simulink model "PMSM_MC_2025a"  (R2025a)
settings: Solver=FixedStepDiscrete  StartTime=0.0  StopTime=10.0  FixedStep=0.00005  RelTol=1e-3
values from neighbouring files (symbols this model uses):
  MC_DCurrLopKi_CFG = 0.008293758    [PMSM_MC_Data_2025a.sldd]
  MC_DCurrLopKp_CFG = 0.0870848    [PMSM_MC_Data_2025a.sldd]
  MC_MotModeDebug_CFG = 255.0    [PMSM_MC_Data_2025a.sldd]
  MC_POLE_NUM_CFG = 7.0    [PMSM_MC_Data_2025a.sldd]
  MC_QCurrLopKi_CFG = 0.008293758    [PMSM_MC_Data_2025a.sldd]
  MC_QCurrLopKp_CFG = 0.0870848    [PMSM_MC_Data_2025a.sldd]
  MC_SpdLopKi_CFG = 1.0E-5    [PMSM_MC_Data_2025a.sldd]
  MC_SpdLopKp_CFG = 0.002    [PMSM_MC_Data_2025a.sldd]
  OpenLoopEn_CFG = 0.0    [PMSM_MC_Data_2025a.sldd]
  SensorLessEn_CFG = 0.0    [PMSM_MC_Data_2025a.sldd]
  SensorLessType_CFG = 1.0    [PMSM_MC_Data_2025a.sldd]
undefined symbols (not defined in the file or in its folder): Ls, magnitude, Rs
libraries: simulink x25, slpidlib x6
(part 3 of 3)

== stateflow chart PMSM_MC_2025a/PMSM_MC/MC_HighFrqTask/OpenLopMod/OpenLopThetaeCal ==
  state Stop
    en:
    //init output
    Thetae_SensLess = 0;
    OLStartCompletedFlag = 0;
    TransmActiveFlag = 0;
    SL_TransferActive = 0;
    //init local variable
    WeRefRamped = 0;
    Thetae_OL = 0;
    OLStableCnt = 0;
    Blend = 0.0F;
    TransmStep = 0;
    TransmFactor = 0;
    DeltaStep  = 0;
    Err = 0;
    RawNow = 0;
    note: 注意要给局部变量
        | 初始化赋值处理
  state VFOpenLoop
    state Align
      en:
      Thetae_SensLess = 0;
    state Open
      en,du:
      Ramping(OLWeRef,OLWeRampMaxStep);
      OLThetaeSum();
      Thetae_SensLess = Thetae_OL;
    (default) -> VFOpenLoop.Align
    VFOpenLoop.Align -> VFOpenLoop.Open : [after(100,msec)]
  state IFStart
    state Align
      en:
      Thetae_SensLess = 0;
    state Open
      en,du:
      Ramping(OLWeRef,OLWeRampMaxStep);
      OLThetaeSum();
      OLStableCntSum();
      Thetae_SensLess = Thetae_OL;
    note: TransmStep其实是根据切换时间算每次
        | 权重增加的步长，最终完成切换从0->1
    state Transm
      en:
      //相位计算与方向判断
      TransmActiveFlag = 1;
      SL_TransferActive = 1;
      Blend  = 0;
      TransmFactor = 0.0F;
      //cal steps according time
      TransmStep = Ts * 1000.0F / OLWeightedTransmTime;
      //transmite from open to close
      WeightedTransmite();
      du:
      WeightedTransmite();
    (default) -> IFStart.Align
    IFStart.Align -> IFStart.Open : [after(100,msec)]
    IFStart.Open -> Transm : [OLStableCnt>OLSpdStableCnt && SL_SpeedReady]
  state Ramping(in,MaxStep) [function]
    note: WeRefRamped指当前的局部真实被电机使用的一个设定递增速度值，电机最开始为0，当我的速度期望值比较大的时候，就会与现在WeRefRamped真实速度设定值比较，让他以MaxStep的递增速度累加或者累减，直到设定值与期望值的差值在[-MaxStep,+MaxStep]时，将当前速度赋值给定成期望值
    (default) -> (junction 23)
    (junction 23) -> (junction 30) [order 1] : [in - WeRefRamped > MaxStep]
    (junction 23) -> (junction 32) [order 2]
    (junction 30) -> (junction 41) : {
        | WeRefRamped = WeRefRamped + MaxStep;
        | }
    (junction 32) -> (junction 34) [order 1] : [in - WeRefRamped < -MaxStep]
    (junction 32) -> (junction 36) [order 2] : {
        | WeRefRamped = in;
        | }
    (junction 34) -> (junction 38) : {
        | WeRefRamped = WeRefRamped - MaxStep;
        | }
    (junction 38) -> (junction 36)
    (junction 41) -> (junction 38)
    (junction 36) -> (junction 43)
  state OLThetaeSum [function]
    note: MotCtrMode==8条件是为了VF开环使用的，
        | 我们的VF开环只进行正向累加，而MotorSpdRef
        | 主要用于IF启动的时候使用
    (default) -> (junction 28)
    (junction 28) -> (junction 48) [order 1] : [MotorSpdRef > 0||...
        | MotCtrMode == 8]
    (junction 28) -> (junction 52) [order 2] : {
        | Thetae_OL = Thetae_OL - WeRefRamped*Ts;
        | }
    (junction 48) -> (junction 50) : {
        | Thetae_OL = Thetae_OL + WeRefRamped*Ts;
        | }
    (junction 50) -> (junction 52)
    (junction 52) -> (junction 55)
    (junction 55) -> (junction 57) [order 1] : [Thetae_OL < 0]
    (junction 55) -> (junction 59) [order 2] : {
        | //set range to [0 2pi]
        | Thetae_OL = fmod(Thetae_OL,6.28318531F);
        | }
    (junction 57) -> (junction 58) : {
        | //set range to [0 2pi]
        | Thetae_OL  = -Thetae_OL;
        | Thetae_OL = fmod(Thetae_OL,6.28318531F);
        | Thetae_OL =  6.28318531F - Thetae_OL;
        | }
    (junction 58) -> (junction 59)
    (junction 59) -> (junction 60)
  state OLStableCntSum [function]
    note: 如果观测器速度大于设定的稳定速度就开始稳定计次
        | 如果出现速度小于阈值则计次再次为0
    (default) -> (junction 79)
    (junction 79) -> (junction 87) [order 1] : [(MotorSpdRef > 0 && We_Est>OLSpdStableThd) ||...
        | (MotorSpdRef < 0 && We_Est<-OLSpdStableThd)]
    (junction 87) -> (junction 85) [order 2]
    (junction 79) -> (junction 85) [order 2] : {
        | OLStableCnt = 0;
        | }
    (junction 87) -> (junction 711) [order 1] : [OLStableCnt <= OLSpdStableCnt]
    (junction 711) -> (junction 86) : {
        | OLStableCnt++;
        | }
    (junction 86) -> (junction 85)
    (junction 85) -> (junction 88)
  state WeightedTransmite_origin [function] [commented out]
    (default) -> (junction 279) [commented out] : {
        | //update factor each sw cycle
        | %TransmFactor = TransmFactor+TransmStep;
        | //open loop angle calculate
        | Ramping(OLWeRef,OLWeRampMaxStep);
        | OLThetaeSum();
        | RawNow = Thetae_Est -Thetae_OL;
        |
        | }
    (junction 279) -> (junction 281) [commented out] : [RawNow>3.1415927F]
    (junction 279) -> (junction 285) [commented out]
    (junction 281) -> (junction 283) [commented out] : {
        | RawNow = RawNow - 6.2831855F;
        | }
    (junction 283) -> (junction 285) [commented out]
    (junction 285) -> (junction 288) [commented out]
    (junction 288) -> (junction 290) [commented out] : [RawNow<-3.1415927F]
    (junction 288) -> (junction 294) [commented out]
    (junction 290) -> (junction 292) [commented out] : {
        | RawNow = RawNow + 6.2831855F;
        | }
    (junction 292) -> (junction 294) [commented out]
    (junction 294) -> (junction 300) [commented out] : {
        | Err = RawNow - PhaseOffset;
        | }
    (junction 300) -> (junction 310) [commented out] : [Err>3.1415927F]
    (junction 300) -> (junction 309) [commented out]
    (junction 310) -> (junction 306) [commented out] : {
        | Err = Err - 6.2831855F;
        | }
    (junction 306) -> (junction 309) [commented out]
    (junction 309) -> (junction 301) [commented out]
    (junction 301) -> (junction 315) [commented out] : [Err<-3.1415927F]
    (junction 301) -> (junction 302) [commented out]
    (junction 315) -> (junction 304) [commented out] : {
        | Err = Err + 6.2831855F;
        | }
    (junction 304) -> (junction 302) [commented out]
    (junction 302) -> (junction 354) [commented out] : {
        | DeltaStep = 0.002f * Err;
        | }
    (junction 354) -> (junction 368) [commented out] : [DeltaStep>0.002F]
    (junction 354) -> (junction 363) [commented out]
    (junction 368) -> (junction 356) [commented out] : {
        | DeltaStep = 0.002F;
        | }
    (junction 356) -> (junction 363) [commented out]
    (junction 363) -> (junction 366) [commented out]
    (junction 366) -> (junction 361) [commented out] : [DeltaStep<-0.002F]
    (junction 366) -> (junction 362) [commented out]
    (junction 361) -> (junction 353) [commented out] : {
        | DeltaStep = -0.002F;
        | }
    (junction 353) -> (junction 362) [commented out]
    (junction 362) -> (junction 336) [commented out] : {
        | //计算最新相位偏差
        | PhaseOffset = PhaseOffset + DeltaStep;
        | }
    (junction 336) -> (junction 350) [commented out] : [PhaseOffset>3.1415927F]
    (junction 336) -> (junction 345) [commented out]
    (junction 350) -> (junction 338) [commented out] : {
        | PhaseOffset = PhaseOffset - 6.2831855F;
        | }
    (junction 338) -> (junction 345) [commented out]
    (junction 345) -> (junction 348) [commented out]
    (junction 348) -> (junction 343) [commented out] : [PhaseOffset<-3.1415927F]
    (junction 348) -> (junction 344) [commented out]
    (junction 343) -> (junction 335) [commented out] : {
        | PhaseOffset = PhaseOffset + 6.2831855F;
        | }
    (junction 335) -> (junction 344) [commented out]
    (junction 344) -> (junction 154) [commented out] : {
        | //计算一下输出的无感模式电角度,要求观测器稳定收敛，
        | //根据权重系数补偿相位差，慢慢从开环角度切换到闭环观测器角度
        | Thetae_SensLess = Thetae_OL +  PhaseOffset;
        | }
    (junction 154) -> (junction 257) [commented out] : [Thetae_SensLess <0]
    (junction 154) -> (junction 262) [commented out]
    (junction 257) -> (junction 259) [commented out] : {
        | //limit to [-PI,PI]
        | Thetae_SensLess  = -Thetae_SensLess;
        | Thetae_SensLess = fmod(Thetae_SensLess,6.28F);
        | Thetae_SensLess =  6.28F - Thetae_SensLess;
        | }
    (junction 259) -> (junction 262) [commented out]
    (junction 262) -> (junction 265) [commented out] : {
        | Thetae_SensLess = fmod(Thetae_SensLess,6.28F);
        | }
    (junction 265) -> (junction 424) [commented out] : {
        | Err = Thetae_Est - Thetae_SensLess;
        | }
    (junction 424) -> (junction 438) [commented out] : [Err>3.1415927F]
    (junction 424) -> (junction 433) [commented out]
    (junction 438) -> (junction 426) [commented out] : {
        | Err = Err - 6.2831855F;
        | }
    (junction 426) -> (junction 433) [commented out]
    (junction 433) -> (junction 436) [commented out]
    (junction 436) -> (junction 431) [commented out] : [Err<-3.1415927F]
    (junction 436) -> (junction 432) [commented out]
    (junction 431) -> (junction 423) [commented out] : {
        | Err = Err + 6.2831855F;
        | }
    (junction 423) -> (junction 432) [commented out]
    (junction 432) -> (junction 373) [commented out]
    (junction 373) -> (junction 380) [commented out] : [Err<0.25&&Err>-0.25]
    (junction 373) -> (junction 381) [commented out] : {
        | TransmFactor = 0;
        | }
    (junction 380) -> (junction 372) [commented out] : {
        | //limit to [0,1]
        | TransmFactor = TransmFactor+1;
        | }
    (junction 372) -> (junction 381) [commented out]
    (junction 381) -> (junction 386) [commented out]
    (junction 386) -> (junction 378) [commented out] : [TransmFactor>2000]
    (junction 386) -> (junction 379) [commented out]
    (junction 378) -> (junction 376) [commented out] : {
        | //开环切闭环完成
        | OLStartCompletedFlag = 1;
        | }
    (junction 376) -> (junction 379) [commented out]
  state WeightedTransmite [function]
    (default) -> (junction 568)
    (junction 568) -> (junction 570) [order 1] : [MotCtrMode == 7]
    (junction 568) -> (junction 572) [order 2]
    (junction 570) -> (junction 578) : {
        | Blend = Blend + TransmStep;
        | }
    (junction 578) -> (junction 572)
    (junction 572) -> (junction 576)
    (junction 576) -> (junction 581) [order 1] : [Blend > 1.0F]
    (junction 576) -> (junction 584) [order 2]
    (junction 581) -> (junction 582) : {
        | Blend = 1.0F;
        | }
    (junction 582) -> (junction 584)
    (junction 584) -> (junction 589) : {
        | RawNow = WeRefRamped;
        | }
    (junction 589) -> (junction 591) [order 1] : [MotorSpdRef < 0]
    (junction 589) -> (junction 595) [order 2]
    (junction 591) -> (junction 593) : {
        | RawNow = -RawNow;
        | }
    (junction 593) -> (junction 595)
    (junction 595) -> (junction 598) : {
        | RawNow = RawNow + Blend * (We_Est - RawNow);
        | Thetae_SensLess = Thetae_SensLess + Ts * RawNow;
        | }
    (junction 598) -> (junction 600) [order 1]
    (junction 600) -> (junction 607) [order 1] : [Thetae_SensLess >= 6.28318531F]
    (junction 598) -> (junction 605) [order 2]
    (junction 600) -> (junction 609) [order 2] : [Thetae_SensLess < 0.0F]
    (junction 607) -> (junction 611) : {
        | Thetae_SensLess =Thetae_SensLess - 6.28318531F;
        | }
    (junction 609) -> (junction 613) : {
        | Thetae_SensLess =Thetae_SensLess + 6.28318531F;
        | }
    (junction 613) -> (junction 605)
    (junction 611) -> (junction 613)
    (junction 605) -> (junction 617)
    (junction 617) -> (junction 619) [order 1] : [Thetae_SensLess >= 6.28318531F ||Thetae_SensLess < 0.0F]
    (junction 617) -> (junction 621) [order 2]
    (junction 619) -> (junction 623) : {
        | Thetae_SensLess = fmod(Thetae_SensLess, 6.28318531F);
        | }
    (junction 623) -> (junction 621)
    (junction 621) -> (junction 626) : {
        | Err = Thetae_Est - Thetae_SensLess;
        | }
    (junction 626) -> (junction 628) [order 1]
    (junction 628) -> (junction 630) [order 1] : [Err > 3.14159265F]
    (junction 626) -> (junction 640) [order 2]
    (junction 628) -> (junction 632) [order 2] : [Err < -3.14159265F]
    (junction 630) -> (junction 634) : {
        | Err = Err - 6.28318531F;
        | }
    (junction 632) -> (junction 636) : {
        | Err = Err + 6.28318531F;
        | }
    (junction 636) -> (junction 640)
    (junction 634) -> (junction 636)
    (junction 640) -> (junction 643) : {
        | DeltaStep = 0.002F * Err;
        | }
    (junction 643) -> (junction 645) [order 1]
    (junction 645) -> (junction 647) [order 1] : [DeltaStep > 0.002F]
    (junction 643) -> (junction 656) [order 2]
    (junction 645) -> (junction 651) [order 2] : [DeltaStep < -0.002F]
    (junction 647) -> (junction 649) : {
        | DeltaStep = 0.002F;
        | }
    (junction 651) -> (junction 653) : {
        | DeltaStep = -0.002F;
        | }
    (junction 653) -> (junction 656)
    (junction 649) -> (junction 653)
    (junction 656) -> (junction 664) : {
        | Thetae_SensLess =Thetae_SensLess + DeltaStep;
        | Err = Err - DeltaStep;
        | }
    (junction 664) -> (junction 665) [order 1]
    (junction 665) -> (junction 670) [order 1] : [Thetae_SensLess >= 6.28318531F]
    (junction 664) -> (junction 663) [order 2]
    (junction 665) -> (junction 676) [order 2] : [Thetae_SensLess < 0.0F]
    (junction 670) -> (junction 677) : {
        | Thetae_SensLess =Thetae_SensLess - 6.28318531F;
        | }
    (junction 676) -> (junction 669) : {
        | Thetae_SensLess =Thetae_SensLess + 6.28318531F;
        | }
    (junction 669) -> (junction 663)
    (junction 677) -> (junction 669)
    (junction 663) -> (junction 679)
    (junction 679) -> (junction 666) [order 1] : [Thetae_SensLess >= 6.28318531F ||Thetae_SensLess < 0.0F]
    (junction 679) -> (junction 684) [order 2]
    (junction 666) -> (junction 681) : {
        | Thetae_SensLess = fmod(Thetae_SensLess, 6.28318531F);
        | }
    (junction 681) -> (junction 684)
    (junction 684) -> (junction 685)
    (junction 685) -> (junction 687) [order 1] : [MotCtrMode == 7]
    (junction 687) -> (junction 689) : [Blend >= 1.0F && SL_SpeedReady && Err > -0.25F && Err < 0.25F]
    (junction 685) -> (junction 697) [order 2] : {
        | TransmFactor = 0.0F;
        | }
    (junction 689) -> (junction 695) : {
        | TransmFactor = TransmFactor + 1.0F;
        | }
    (junction 695) -> (junction 697)
    (junction 697) -> (junction 700)
    (junction 700) -> (junction 702) [order 1] : [TransmFactor >= 2000.0F]
    (junction 700) -> (junction 706) [order 2]
    (junction 702) -> (junction 704) : {
        | OLStartCompletedFlag = true;
        | }
    (junction 704) -> (junction 706)
  note: 加上MotCtrMode == 5条件判断的原因是由于速度环和电流环切换时序不一样，模式切换在低频任务中，为避免速度环和速度环积分影响，需要双条件判断
  state CloseLop
    en:
    TransmActiveFlag = 0;
    SL_TransferActive = 0;
    Blend = 1.0F;
    WeightedTransmite();
    du:
    WeightedTransmite();
  (default) -> Stop
  Stop -> VFOpenLoop [order 1] : [MotCtrMode==8]
  VFOpenLoop -> Stop : [MotCtrMode!=8]
  Stop -> IFStart [order 2] : [MotCtrMode==7]
  IFStart -> Stop [order 2] : [MotCtrMode != 7 &&...
      |  !(OLStartCompletedFlag && MotCtrMode == 5)]
  CloseLop -> Stop : [MotCtrMode!=5]
  IFStart -> CloseLop [order 1] : [OLStartCompletedFlag==1&&...
      | MotCtrMode==5]
  data: in function_input single; MaxStep function_input single; MotCtrMode input uint8; We_Est input single; Thetae_Est input single; MotorSpdRef input int16; OLWeRef input single; OLWeRampMaxStep input single; OLSpdStableThd input single; OLSpdStableCnt input single; Ts input single; Thetae_SensLess output single; OLStartCompletedFlag output boolean; WeRefRamped local single; OLWeightedTransmTime input single; Thetae_OL local single; OLStableCnt local uint16; TransmStep local single; TransmFactor local single; Blend local single; Err local single; RawNow local single; DeltaStep local single; TransmActiveFlag output boolean; SL_TransferActive data_store_memory; SL_SpeedReady data_store_memory
